simulink model "matrix_riccati"  (Simulink 5.0)
settings: Solver=ode5  StartTime=0.0  StopTime=20  RelTol=1e-3
values from neighbouring files (symbols this model uses):
  F = [0  1; -0.9  -0.8]    [harmosc_ricatti.mat]    (also in harmosc_riccati.mat; lec.m = ones(n,1); state9.m = [ 0     rho_z  -rho_y     1     0     0     0     0     0; state9_01.mat = [0 0 -7.85492378154e-07 -1.53754144823e-06 0 0 0 0 0 0 0 -7.)
  H = [1 0]    [constant_velocity.m]    (also in damposc.m; harmosc_ricatti.mat; harmosc_riccati.mat; kf_resistor_demo.m = 1)
  P0 = [0.01 0; 0 0.01]    [constant_velocity.m]    (also in damposc.m; harmosc_ricatti.mat = [0.95  0; 0  1]; harmosc_riccati.mat = [1  0; 0  1]; kalgen.m = proc_noise * eye(n))
  Q = [0.0001 0; 0 0.000001]    [constant_velocity.m]    (also in damposc.m = [0.00001 0; 0 0.000001]; harmosc_ricatti.mat = [1  0; 0  1]; harmosc_riccati.mat = [1  0; 0  1]; kalgen.m = proc_noise * eye(n))
  R = Re + h    (= 6378441.8)    [Ainit.m]    (also in constant_velocity.m = 1; damposc.m = 0.01; harmosc_ricatti.mat = 2; harmosc_riccati.mat = 3)
settings Model: Creator=mcarroll  LastModifiedBy=mcarroll  ExtModeAutoUpdateStatusClock=off  SaveFormat=StructureWithTime

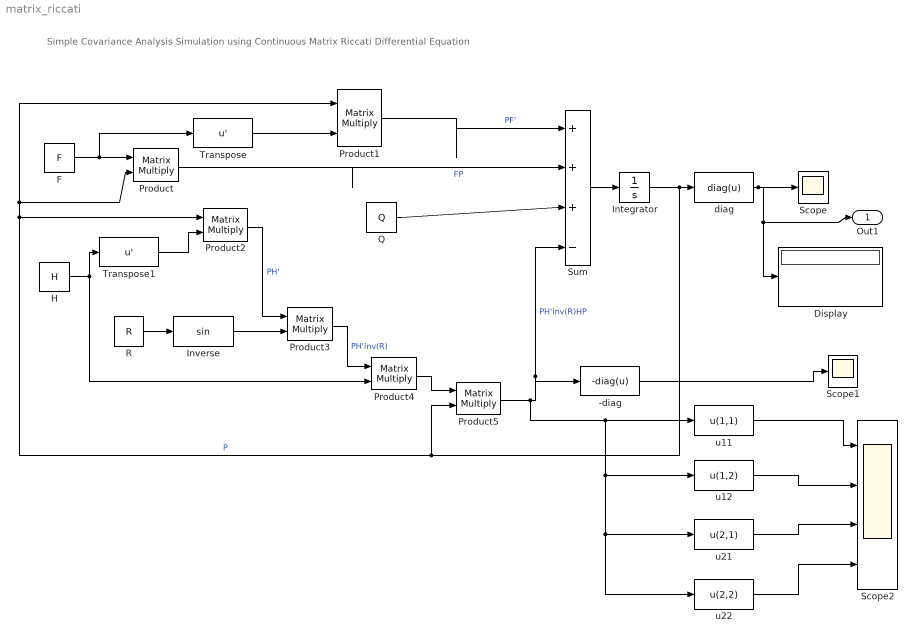
== system matrix_riccati ==
  note: Simple Covariance Analysis Simulation
      | using
      | Continuous Matrix Riccati Differential  Equation
  -diag : MATLABFcn  MATLABFcn=-diag(u)  Output1D=off
  Display : Display
  F : Constant  Value=F  VectorParams1D=off
  H : Constant  Value=H  VectorParams1D=off
  Integrator : Integrator  InitialCondition=P0
  Inverse : MATLABFcn  Output1D=off
  Product{,1..5} (6 alike) : Product  Multiplication=Matrix(*)  SaturateOnIntegerOverflow=on
  Q : Constant  Value=Q  VectorParams1D=off
  R : Constant  Value=R  VectorParams1D=off
  Scope : Scope
      settings: TimeRange=10  YMin=0.8  YMax=2.6
  Scope1 : Scope
      settings: YMin=0  YMax=650
  Scope2 : Scope  NumInputPorts=4
      settings: YMin=0~-5~-5~-5  YMax=650~5~5~5  SaveName=ScopeData2
  Sum : Sum  Inputs=|+++-  SaturateOnIntegerOverflow=on
  Transpose : MATLABFcn  MATLABFcn=u'  Output1D=off
  Transpose1 : MATLABFcn  MATLABFcn=u'  Output1D=off
  diag : MATLABFcn  MATLABFcn=diag(u)  Output1D=off
  u11 : MATLABFcn  MATLABFcn=u(1,1)  Output1D=off
  u12 : MATLABFcn  MATLABFcn=u(1,2)  Output1D=off
  u21 : MATLABFcn  MATLABFcn=u(2,1)  Output1D=off
  u22 : MATLABFcn  MATLABFcn=u(2,2)  Output1D=off
  Out1 : Outport
  wires:
  Integrator/1 -> Product/2, Product1/1, Product2/1, Product5/2, diag/1  "P"
  F/1 -> Product/1, Transpose/1
  Transpose/1 -> Product1/2
  Q/1 -> Sum/3
  H/1 -> Transpose1/1, Product4/2
  Transpose1/1 -> Product2/2
  R/1 -> Inverse/1
  Product2/1 -> Product3/1  "PH'"
  Inverse/1 -> Product3/2
  Product3/1 -> Product4/1  "PH'inv(R)"
  Product4/1 -> Product5/1
  Sum/1 -> Integrator/1
  Product5/1 -> Sum/4, -diag/1, u11/1, u12/1, u21/1, u22/1  "PH'inv(R)HP"
  Product1/1 -> Sum/1  "PF'"
  Product/1 -> Sum/2  "FP"
  diag/1 -> Scope/1, Display/1, Out1/1
  -diag/1 -> Scope1/1
  u11/1 -> Scope2/1
  u22/1 -> Scope2/4
  u21/1 -> Scope2/3
  u12/1 -> Scope2/2
